simulink model "NonlinearModelNorm"  (R2026b)
settings: Solver=VariableStepAuto
undefined symbols (not defined in the file): nom, p_a, p_m
settings Model: Creator=User  LastModifiedBy=User

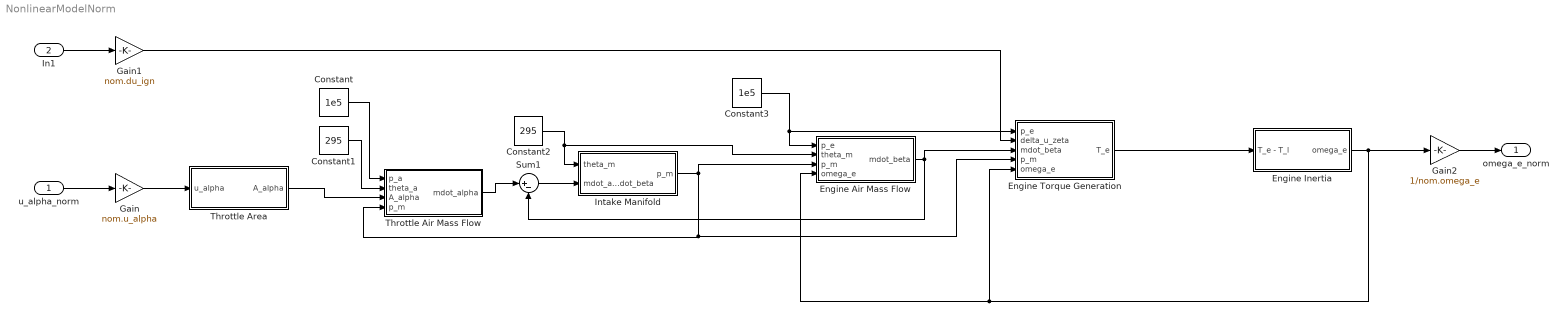
== system NonlinearModelNorm ==
  u_alpha_norm : Inport
  In1 : Inport  Port=2
  Constant : Constant  Value=1e5
  Constant1 : Constant  Value=295
  Constant2 : Constant  Value=295
  Constant3 : Constant  Value=1e5
  Engine Air Mass Flow : Subsystem
  Engine Inertia : Subsystem
  Engine Torque Generation : Subsystem
  Gain : Gain  Gain=nom.u_alpha
  Gain1 : Gain  Gain=nom.du_ign
  Gain2 : Gain  Gain=1/nom.omega_e
  Intake Manifold : Subsystem
  Sum1 : Sum  Inputs=|+-
  Throttle Air Mass Flow : Subsystem
  Throttle Area : Subsystem
  omega_e_norm : Outport
  wires:
  u_alpha_norm/1 -> Gain/1
  Engine Inertia/1(omega_e) -> Gain2/1, Engine Torque Generation/5(omega_e), Engine Air Mass Flow/4(omega_e)
  Constant3/1 -> Engine Torque Generation/1(p_e), Engine Air Mass Flow/1(p_e)
  Throttle Area/1(A_alpha) -> Throttle Air Mass Flow/3(A_alpha)
  Constant/1 -> Throttle Air Mass Flow/1(p_a)
  Constant1/1 -> Throttle Air Mass Flow/2(theta_a)
  Sum1/1 -> Intake Manifold/2(mdot_alpha-mdot_beta)
  Constant2/1 -> Engine Air Mass Flow/2(theta_m), Intake Manifold/1(theta_m)
  Engine Torque Generation/1(T_e) -> Engine Inertia/1(T_e - T_l)
  Throttle Air Mass Flow/1(mdot_alpha) -> Sum1/1
  Intake Manifold/1(p_m) -> Engine Air Mass Flow/3(p_m), Engine Torque Generation/4(p_m), Throttle Air Mass Flow/4(p_m)
  Engine Air Mass Flow/1(mdot_beta) -> Engine Torque Generation/3(mdot_beta), Sum1/2
  Gain/1 -> Throttle Area/1(u_alpha)
  In1/1 -> Gain1/1
  Gain1/1 -> Engine Torque Generation/2(delta_u_zeta)
  Gain2/1 -> omega_e_norm/1

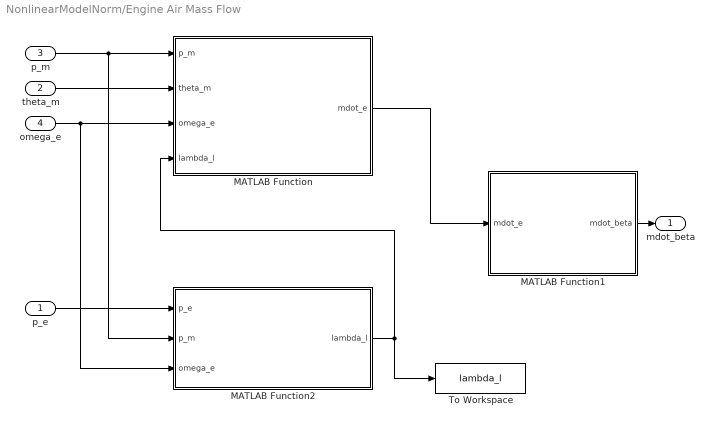
== system NonlinearModelNorm/Engine Air Mass Flow ==
  p_e : Inport
  theta_m : Inport  Port=2
  p_m : Inport  Port=3
  omega_e : Inport  Port=4
  MATLAB Function : MATLAB Function  TreatAsAtomicUnit=on
  MATLAB Function1 : MATLAB Function  TreatAsAtomicUnit=on
  MATLAB Function2 : MATLAB Function  TreatAsAtomicUnit=on
  To Workspace : ToWorkspace  VariableName=lambda_l  SaveFormat=Timeseries  SampleTime=-1
  mdot_beta : Outport
  wires:
  MATLAB Function2/1(lambda_l) -> MATLAB Function/4(lambda_l), To Workspace/1
  MATLAB Function1/1(mdot_beta) -> mdot_beta/1
  theta_m/1 -> MATLAB Function/2(theta_m)
  p_e/1 -> MATLAB Function2/1(p_e)
  p_m/1 -> MATLAB Function2/2(p_m), MATLAB Function/1(p_m)
  MATLAB Function/1(mdot_e) -> MATLAB Function1/1(mdot_e)
  omega_e/1 -> MATLAB Function/3(omega_e), MATLAB Function2/3(omega_e)

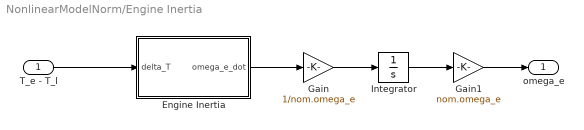
== system NonlinearModelNorm/Engine Inertia ==
  T_e - T_l : Inport
  Engine Inertia : MATLAB Function  TreatAsAtomicUnit=on
  Gain : Gain  Gain=1/nom.omega_e
  Gain1 : Gain  Gain=nom.omega_e
  Integrator : Integrator  InitialCondition=1
  omega_e : Outport
  wires:
  T_e - T_l/1 -> Engine Inertia/1(delta_T)
  Integrator/1 -> Gain1/1
  Engine Inertia/1(omega_e_dot) -> Gain/1
  Gain/1 -> Integrator/1
  Gain1/1 -> omega_e/1

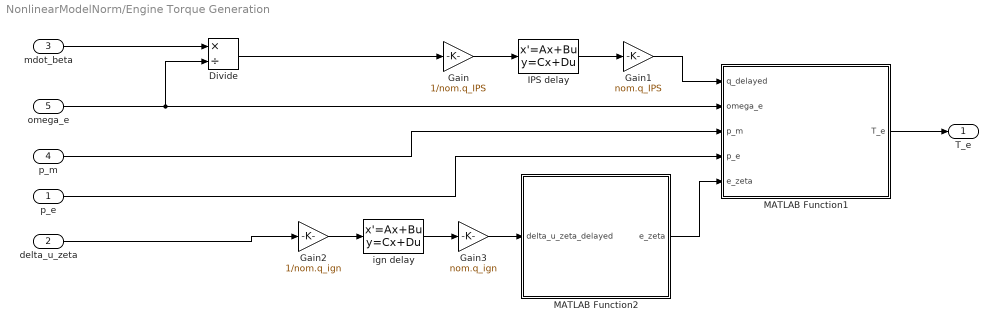
== system NonlinearModelNorm/Engine Torque Generation ==
  p_e : Inport
  delta_u_zeta : Inport  Port=2
  mdot_beta : Inport  Port=3
  p_m : Inport  Port=4
  omega_e : Inport  Port=5
  Divide : Product  Inputs=*/
  Gain : Gain  Gain=1/nom.q_IPS
  Gain1 : Gain  Gain=nom.q_IPS
  Gain2 : Gain  Gain=1/nom.q_ign
  Gain3 : Gain  Gain=nom.q_ign
  IPS delay : StateSpace  A=nom.Aips  B=nom.Bips  C=nom.Cips  D=nom.Dips  InitialCondition=nom.x0ips
  MATLAB Function1 : MATLAB Function  TreatAsAtomicUnit=on
  MATLAB Function2 : MATLAB Function  TreatAsAtomicUnit=on
  ign delay : StateSpace  A=nom.Aign  B=nom.Bign  C=nom.Cign  D=nom.Dign  InitialCondition=nom.x0ign
  T_e : Outport
  wires:
  p_m/1 -> MATLAB Function1/3(p_m)
  delta_u_zeta/1 -> Gain2/1
  omega_e/1 -> MATLAB Function1/2(omega_e), Divide/2
  MATLAB Function1/1(T_e) -> T_e/1
  mdot_beta/1 -> Divide/1
  IPS delay/1 -> Gain1/1
  MATLAB Function2/1(e_zeta) -> MATLAB Function1/5(e_zeta)
  p_e/1 -> MATLAB Function1/4(p_e)
  ign delay/1 -> Gain3/1
  Divide/1 -> Gain/1
  Gain/1 -> IPS delay/1
  Gain1/1 -> MATLAB Function1/1(q_delayed)
  Gain2/1 -> ign delay/1
  Gain3/1 -> MATLAB Function2/1(delta_u_zeta_delayed)

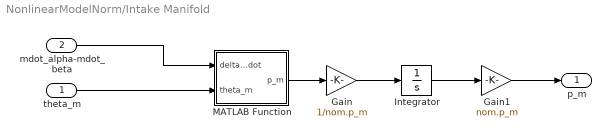
== system NonlinearModelNorm/Intake Manifold ==
  theta_m : Inport
  mdot_alpha-mdot_beta : Inport  Port=2
  Gain : Gain  Gain=1/nom.p_m
  Gain1 : Gain  Gain=nom.p_m
  Integrator : Integrator  InitialCondition=1
  MATLAB Function : MATLAB Function  TreatAsAtomicUnit=on
  p_m : Outport
  wires:
  Integrator/1 -> Gain1/1
  mdot_alpha-mdot_beta/1 -> MATLAB Function/1(delta_mdot)
  theta_m/1 -> MATLAB Function/2(theta_m)
  MATLAB Function/1(p_m) -> Gain/1
  Gain/1 -> Integrator/1
  Gain1/1 -> p_m/1

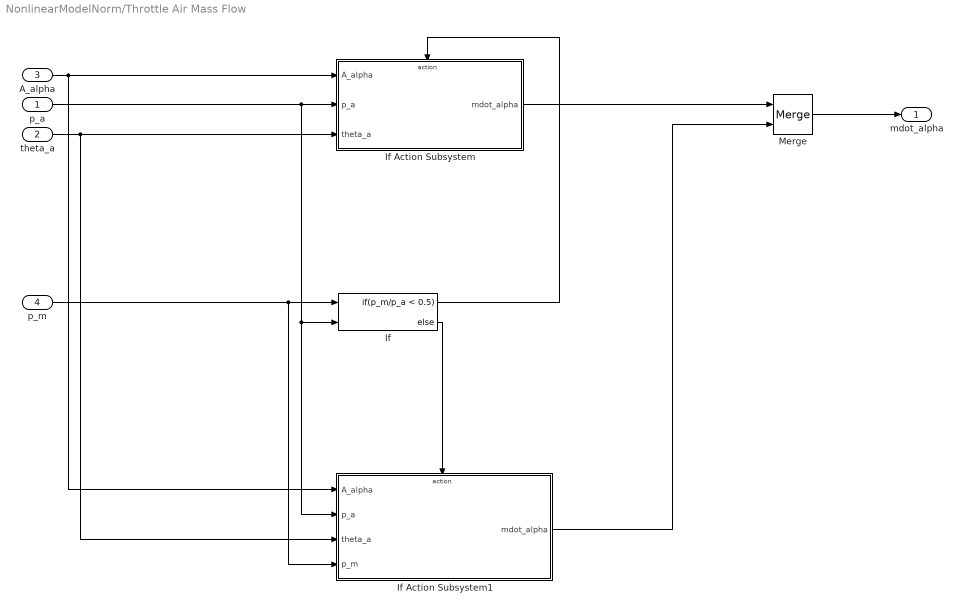
== system NonlinearModelNorm/Throttle Air Mass Flow ==
  p_a : Inport
  theta_a : Inport  Port=2
  A_alpha : Inport  Port=3
  p_m : Inport  Port=4
  If : If  NumInputs=2  IfExpression=p_m/p_a < 0.5  InportLabels=p_m,p_a
  If Action Subsystem : Subsystem  TreatAsAtomicUnit=on
  If Action Subsystem1 : Subsystem  TreatAsAtomicUnit=on
  Merge : Merge
  mdot_alpha : Outport
  wires:
  theta_a/1 -> If Action Subsystem/3(theta_a), If Action Subsystem1/3(theta_a)
  Merge/1 -> mdot_alpha/1
  If Action Subsystem/1(mdot_alpha) -> Merge/1
  p_a/1 -> If/2, If Action Subsystem1/2(p_a), If Action Subsystem/2(p_a)
  A_alpha/1 -> If Action Subsystem/1(A_alpha), If Action Subsystem1/1(A_alpha)
  If/2 -> If Action Subsystem1/Action
  If Action Subsystem1/1(mdot_alpha) -> Merge/2
  p_m/1 -> If/1, If Action Subsystem1/4(p_m)
  If/1 -> If Action Subsystem/Action

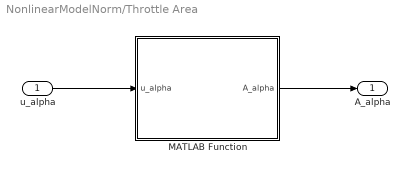
== system NonlinearModelNorm/Throttle Area ==
  u_alpha : Inport
  MATLAB Function : MATLAB Function  TreatAsAtomicUnit=on
  A_alpha : Outport
  wires:
  u_alpha/1 -> MATLAB Function/1(u_alpha)
  MATLAB Function/1(A_alpha) -> A_alpha/1

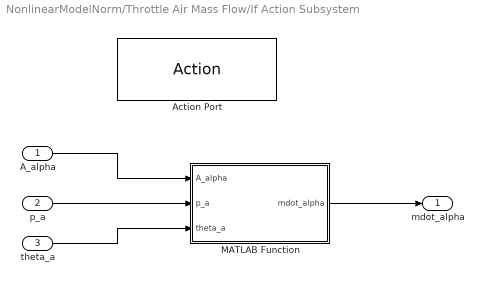
== system NonlinearModelNorm/Throttle Air Mass Flow/If Action Subsystem ==
  A_alpha : Inport
  p_a : Inport  Port=2
  theta_a : Inport  Port=3
  Action Port : ActionPort  ActionPortLabel=if(p_m/p_a < 0.5)
  MATLAB Function : MATLAB Function  TreatAsAtomicUnit=on
  mdot_alpha : Outport
  wires:
  A_alpha/1 -> MATLAB Function/1(A_alpha)
  p_a/1 -> MATLAB Function/2(p_a)
  theta_a/1 -> MATLAB Function/3(theta_a)
  MATLAB Function/1(mdot_alpha) -> mdot_alpha/1

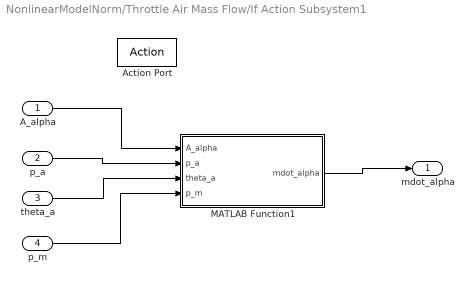
== system NonlinearModelNorm/Throttle Air Mass Flow/If Action Subsystem1 ==
  A_alpha : Inport
  p_a : Inport  Port=2
  theta_a : Inport  Port=3
  p_m : Inport  Port=4
  Action Port : ActionPort  ActionPortLabel=else
  MATLAB Function1 : MATLAB Function  TreatAsAtomicUnit=on
  mdot_alpha : Outport
  wires:
  A_alpha/1 -> MATLAB Function1/1(A_alpha)
  p_a/1 -> MATLAB Function1/2(p_a)
  theta_a/1 -> MATLAB Function1/3(theta_a)
  p_m/1 -> MATLAB Function1/4(p_m)
  MATLAB Function1/1(mdot_alpha) -> mdot_alpha/1

== matlab function NonlinearModelNorm/Engine Air Mass Flow/MATLAB Function2 ==
  data: p_e input; lambda_l output; p_m input; omega_e input; params parameter
function lambda_l = VolumetricEfficiency(p_e, p_m, omega_e, params)

% Volumetric efficiency

lambda_lp = (params.V_c + params.V_d)/params.V_d ...
            - params.V_c/params.V_d ...
            * (p_e/p_m)^(1/params.kappa);

lambda_lomega = params.gamma_0 + params.gamma_1 * omega_e;

lambda_l = lambda_lp * lambda_lomega;

end

== matlab function NonlinearModelNorm/Intake Manifold/MATLAB Function ==
  data: delta_mdot input; theta_m input; p_m output; params parameter
function p_m = fcn(delta_mdot, theta_m, params)

p_m = delta_mdot * theta_m * params.R / params.Vm;

== matlab function NonlinearModelNorm/Throttle Air Mass Flow/If Action Subsystem/MATLAB Function ==
  data: A_alpha input; mdot_alpha output; p_a input; theta_a input; params parameter
function mdot_alpha = fcn(A_alpha,p_a,theta_a, params)

mdot_alpha = A_alpha * p_a/sqrt(params.R*theta_a) * 1/sqrt(2);

== matlab function NonlinearModelNorm/Throttle Air Mass Flow/If Action Subsystem1/MATLAB Function1 ==
  data: A_alpha input; mdot_alpha output; p_a input; theta_a input; p_m input; params parameter
function mdot_alpha = fcn(A_alpha, p_a, theta_a, p_m, params)

% if p_m/p_a >=1
%     mdot_alpha = 1;
%     fprintf('\nratio greater 1')
% else
%     mdot_alpha = A_alpha * p_a / sqrt(params.R * theta_a) * sqrt((2*p_m/p_a)*(1-p_m/p_a));
% end

mdot_alpha = A_alpha * p_a / sqrt(params.R * theta_a) * sqrt((2*p_m/p_a)*(1-p_m/p_a));

== matlab function NonlinearModelNorm/Engine Inertia/Engine Inertia ==
  data: delta_T input; omega_e_dot output; params parameter
function omega_e_dot = fcn(delta_T, params)

omega_e_dot = (1/params.theta_e)*(delta_T);

== matlab function NonlinearModelNorm/Engine Torque Generation/MATLAB Function1 ==
  data: q_delayed input double; omega_e input double; p_m input double; p_e input double; e_zeta input double; params parameter; T_e output double
function T_e = EngineTorque(q_delayed, omega_e, p_m, p_e, e_zeta, params)

% Torque produced by the engine

e_p_mphi = (params.eta_0 + params.eta_1*omega_e) ...
           * e_zeta * params.H_l/params.V_d ...
           * 4*pi/(params.lambda*params.sigma_0) ...
           * q_delayed;

p_me0f = params.beta_0 * 4*pi/params.V_d;

p_me0g = p_e - p_m;

p_me = e_p_mphi - p_me0f - p_me0g;

T_e = p_me * params.V_d/(4*pi);


end

== matlab function NonlinearModelNorm/Engine Torque Generation/MATLAB Function2 ==
  data: delta_u_zeta_delayed input; e_zeta output; params parameter
function e_zeta = IgnitionEfficiency(delta_u_zeta_delayed, params)

e_zeta = 1 - params.k_zeta * delta_u_zeta_delayed^2;

end

== matlab function NonlinearModelNorm/Throttle Area/MATLAB Function ==
  data: u_alpha input; A_alpha output; params parameter
function A_alpha = fcn(u_alpha, params)

A_alpha = params.alpha_0 + params.alpha_1*u_alpha;

== matlab function NonlinearModelNorm/Engine Air Mass Flow/MATLAB Function ==
  data: mdot_e output; p_m input; theta_m input; omega_e input; lambda_l input; params parameter
function mdot_e = FreshMixtureMassFlow(p_m, theta_m, omega_e, lambda_l, params)

% Fresh mixture that enters the cylinder

mdot_e = 1/2 ... 
         * p_m/(params.R*theta_m) ...
         * lambda_l ...
         * params.V_d ... 
         * omega_e/(2*pi);

end

== matlab function NonlinearModelNorm/Engine Air Mass Flow/MATLAB Function1 ==
  data: mdot_beta output; mdot_e input; params parameter
function mdot_beta = MixtureToAirMassFlow(mdot_e, params)

% Air mass flow out of the intake manifold

mdot_beta = mdot_e / (1 + (1 / (params.lambda * params.sigma_0)));

end
